simulink model "CNC_pp_obs"  (R2024b)
settings: Solver=VariableStepAuto  StartTime=0.0  StopTime=10.0  RelTol=1e-3
PostLoadFcn:
  | addpath(fileparts(fileparts(get_param(bdroot,'FileName'))));
StartFcn:
  |    addpath(fullfile(fileparts(get_param(bdroot,'FileName')),'..','scripts'));
  |    run_and_save_deferred(bdroot, 'start');
StopFcn:
  |    addpath(fullfile(fileparts(get_param(bdroot,'FileName')),'..','scripts'));
  |    run_and_save_deferred(bdroot, 'stop');
undefined symbols (not defined in the file): A_obs_3165, A_obs_3166, B_obs_3165, B_obs_3166, HIL, k_3165_load, k_3166_load, Kaw_3165, Kaw_3166, kd_3165, kd_3166, ki_3165, Ki_3165, ki_3166, Ki_3166, kp_3165, kp_3166, Kx_3165, Kx_3166, qc_get_step_size, tau_3165_load, tau_3166_load
libraries: quarc_library x4, slpidlib x2
settings Model: Creator=ricca  LastModifiedBy=ricca

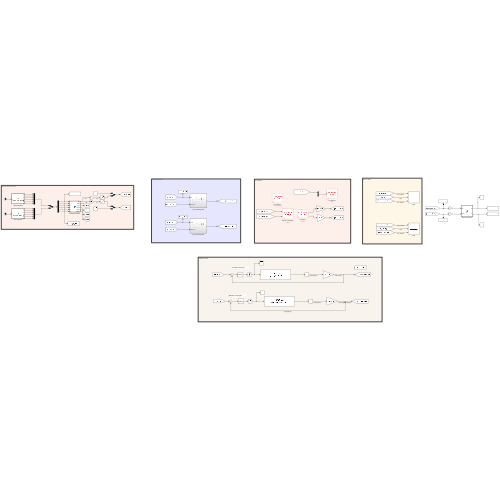
[thumbnail: Simulink's stored preview of the top-level diagram]
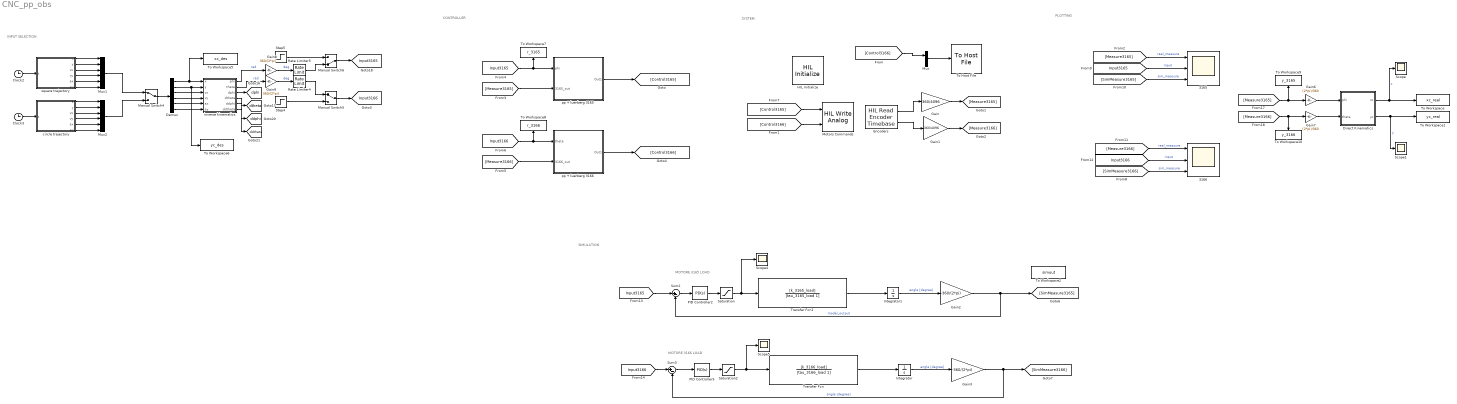
== system CNC_pp_obs ==
  note: MOTORE 3165 LOAD
  note: PLOTTING
  note: CONTROLLER
  note: MOTORE 3166 LOAD
  note: SIMULATION
  note: SYSTEM
  note: INPUT SELECTION
  3165 : Scope  NumInputPorts=3
  3166 : Scope  NumInputPorts=3
  Clock2 : Clock
  Clock3 : Clock
  Demux : Demux  Outputs=6
  Direct Kinematics : MATLAB Function  TreatAsAtomicUnit=on  SystemSampleTime=0.002
  Encoders : quarc_library/Data Acquisition/Generic/Timebases/HIL Read Encoder Timebase  object_name=HIL-1  clock=0  channels=0:1  active=on  vector_output=off  data_type_mode=Inherit via back propagation  data_type=double  overflow_mode=Error on overflow  samples_in_buffer=max(ceil(1/qc_get_step_size), 1)
  Gain : Gain  Gain=360/4096
  Gain1 : Gain  Gain=360/4096
  Gain2 : Gain  Gain=-360/(2*pi)
  Gain3 : Gain  Gain=-360/(2*pi)
  Gain6 : Gain  Gain=(2*pi)/360
  Gain7 : Gain  Gain=(2*pi)/360
  Gain8 : Gain  Gain=360/(2*pi)
  Gain9 : Gain  Gain=360/(2*pi)
  HIL Initialize : quarc_library/Data Acquisition/Generic/Configuration/HIL Initialize  object_name=HIL-1  board_type=q2_usb  board_number=0  board_options=d0=digital;d1=digital;led=auto;update_rate=normal;decimation=1  exclusive=off  active=off  hardware_clocks=[0]  clock_modes=[]  initial_clock_frequencies=[]  set_clock_params_at_start=off  set_clock_params_at_switch_in=off  set_clock_frequencies_at_start=off  set_clock_frequencies_at_switch_in=off  analog_input_channels=[0:1]  analog_input_configurations=[]  analog_input_maximums=10  analog_input_minimums=-10  set_analog_input_params_at_start=on  set_analog_input_params_at_switch_in=off  analog_output_channels=[0:1]  analog_output_maximums=10  analog_output_minimums=-10  initial_analog_outputs=[0]  final_analog_outputs=[0]  watchdog_analog_outputs=0  set_analog_output_params_at_start=on  set_analog_output_params_at_switch_in=off  set_analog_outputs_at_start=on  set_analog_outputs_at_switch_in=off  set_analog_outputs_at_terminate=on  set_analog_outputs_at_switch_out=off  set_analog_outputs_on_watchdog=off  digital_input_channels=[]  digital_output_channels=[]  digital_output_configuration=[]  initial_digital_outputs=[1]  final_digital_outputs=[1]  watchdog_digital_outputs=[1]  set_digital_output_params_at_start=off  set_digital_output_params_at_switch_in=off  set_digital_outputs_at_start=on  set_digital_outputs_at_switch_in=off  set_digital_outputs_at_terminate=on  set_digital_outputs_at_switch_out=off  set_digital_outputs_on_watchdog=off  encoder_channels=[0:1]  quadrature=[4]  encoder_filter_frequency=[]  initial_encoder_counts=[0]  set_encoder_params_at_start=on  set_encoder_params_at_switch_in=off  set_encoder_counts_at_start=on  set_encoder_counts_at_switch_in=off  pwm_channels=[]  pwm_modes=[0]  pwm_frequency=1/0.020  pwm_configuration=[]  pwm_alignment=[]  pwm_polarity=[]  pwm_leading_deadband=[]  pwm_trailing_deadband=[]  initial_pwm_outputs=[0]  final_pwm_outputs=[0]  watchdog_pwm_outputs=[0]  set_pwm_params_at_start=on  set_pwm_params_at_switch_in=off  set_pwm_outputs_at_start=on  set_pwm_outputs_at_switch_in=off  set_pwm_outputs_at_terminate=on  set_pwm_outputs_at_switch_out=off  set_pwm_outputs_on_watchdog=off  other_output_channels=[]  initial_other_outputs=[]  final_other_outputs=[]  watchdog_other_outputs=[]  set_other_outputs_at_start=off  set_other_outputs_at_switch_in=off  set_other_outputs_at_terminate=off  set_other_outputs_at_switch_out=off  set_other_outputs_on_watchdog=off
  Integrator : Integrator
  Integrator1 : Integrator
  Manual Switch4 : ManualSwitch
  Manual Switch5 : ManualSwitch
  Manual Switch6 : ManualSwitch  CurrentSetting=0
  Motors Commands : quarc_library/Data Acquisition/Generic/Immediate I//O/HIL Write Analog  object_name=HIL-1  channels=0:1  sample_time=-1  active=off  vector_input=off
  Mux : Mux  Inputs=2
  Mux1 : Mux  Inputs=6
  Mux2 : Mux  Inputs=6
  PID Controller2 : slpidlib/PID Controller  Controller=PD  Form=Parallel  TimeDomain=Continuous-time  UseExternalTs=off  SampleTime=-1  IntegratorMethod=Forward Euler  FilterMethod=Forward Euler  ControllerParametersSource=internal  P=kp_3165  I=ki_3165  UseKiTs=off  D=kd_3165  UseExternalDerivativeSource=off  N=100  UseFilter=on  TunerSelectOption=Transfer Function Based (PID Tuner App)  InitialConditionSource=internal  InitialConditionForIntegrator=0  InitialConditionForFilter=0  DifferentiatorICPrevScaledInput=0  ExternalReset=none  TrackingMode=off  Kt=1  LimitOutput=off  SatLimitsSource=internal  UpperSaturationLimit=inf  LowerSaturationLimit=-inf  LinearizeAsGain=on  AntiWindupMode=none  Kb=1  LimitIntegrator=off  UpperIntegratorSaturationLimit=inf  LowerIntegratorSaturationLimit=-inf  POutMin=[]  POutMax=[]  IOutMin=[]  IOutMax=[]  DOutMin=[]  DOutMax=[]  NOutMin=[]  NOutMax=[]  SumOutMin=[]  SumOutMax=[]  SaturationOutMin=[]  SaturationOutMax=[]  PParamMin=[]  PParamMax=[]  IParamMin=[]  IParamMax=[]  DParamMin=[]  DParamMax=[]  NParamMin=[]  NParamMax=[]  KbParamMin=[]  KbParamMax=[]  KtParamMin=[]  KtParamMax=[]  KbOutMin=[]  KbOutMax=[]  KtOutMin=[]  KtOutMax=[]  IntegratorOutMin=[]  IntegratorOutMax=[]  FilterOutMin=[]  FilterOutMax=[]  SumI1OutMin=[]  SumI1OutMax=[]  SumI2OutMin=[]  SumI2OutMax=[]  SumI3OutMin=[]  SumI3OutMax=[]  SumI4OutMin=[]  SumI4OutMax=[]  SumDOutMin=[]  SumDOutMax=[]  DifferentiatorOutMin=[]  DifferentiatorOutMax=[]  FilterDiffOutCoefMin=[]  FilterDiffOutCoefMax=[]  ReciprocalOutMin=[]  ReciprocalOutMax=[]  SumDenOutMin=[]  SumDenOutMax=[]  SumNumOutMin=[]  SumNumOutMax=[]  DivideOutMin=[]  DivideOutMax=[]  UdiffTsProdOutMin=[]  UdiffTsProdOutMax=[]  NTsProdOutMin=[]  NTsProdOutMax=[]  UintegralTsProdOutMin=[]  UintegralTsProdOutMax=[]  UngainTsProdOutMin=[]  UngainTsProdOutMax=[]  ClampingZeroOutDataTypeStr=Inherit: Inherit via back propagation  ClampingZeroOutMin=[]  ClampingZeroOutMax=[]  FilterDenConstantOutDataTypeStr=Inherit: Inherit via back propagation  FilterDenConstantOutMin=[]  FilterDenConstantOutMax=[]  PCopyOutDataTypeStr=Inherit: Inherit via back propagation  PCopyOutMin=[]  PCopyOutMax=[]  NCopyOutDataTypeStr=Inherit: Inherit via back propagation  NCopyOutMin=[]  NCopyOutMax=[]  IntegratorContinuousStateAttributes=''  IntegratorStateMustResolveToSignalObject=off  IntegratorRTWStateStorageClass=Auto  FilterContinuousStateAttributes=''  FilterStateMustResolveToSignalObject=off  FilterRTWStateStorageClass=Auto  ParallelPVariant=InternalParameters  IdealPVariant=Disabled  IVariant=Disabled  DVariant=InternalParameters  IntegratorVariant=Disabled  SatVariant=Disabled  AWVariant=Disabled  PCopyVariant=Disabled  TRVariant=Disabled  FdbkBlocksVariant=Forward  IdealPFdbkVariant=Disabled  SatFdbkVariant=Disabled  DerivativeFilterVariant=ContFilter  NVariant=InternalParameters  NCopyVariant=Disabled  FilterICVariant=InternalICsFilter  IntegratorICVariant=Disabled  ExternalResetVariant=Disabled  TRSumVariant=Passthrough  SumFdbkVariant=Disabled  SumVariant=Sum_PD  TsampFilterVariant=InternalTs  TsampNgainVariant=Passthrough  TsampIntegralVariant=Disabled_SignalSpec  ExternalSaturationOutDataTypeStr=Inherit: Same as second input  DerivativeSourceVariant=ErrorSignal  PreIntVariant=InternalPreInt
  PID Controller3 : slpidlib/PID Controller  Controller=PID  Form=Parallel  TimeDomain=Continuous-time  UseExternalTs=off  SampleTime=-1  IntegratorMethod=Forward Euler  FilterMethod=Forward Euler  ControllerParametersSource=internal  P=kp_3166  I=ki_3166  UseKiTs=off  D=kd_3166  UseExternalDerivativeSource=off  N=100  UseFilter=on  TunerSelectOption=Transfer Function Based (PID Tuner App)  InitialConditionSource=internal  InitialConditionForIntegrator=0  InitialConditionForFilter=0  DifferentiatorICPrevScaledInput=0  ExternalReset=none  TrackingMode=off  Kt=1  LimitOutput=off  SatLimitsSource=internal  UpperSaturationLimit=inf  LowerSaturationLimit=-inf  LinearizeAsGain=on  AntiWindupMode=none  Kb=1  LimitIntegrator=off  UpperIntegratorSaturationLimit=inf  LowerIntegratorSaturationLimit=-inf  POutMin=[]  POutMax=[]  IOutMin=[]  IOutMax=[]  DOutMin=[]  DOutMax=[]  NOutMin=[]  NOutMax=[]  SumOutMin=[]  SumOutMax=[]  SaturationOutMin=[]  SaturationOutMax=[]  PParamMin=[]  PParamMax=[]  IParamMin=[]  IParamMax=[]  DParamMin=[]  DParamMax=[]  NParamMin=[]  NParamMax=[]  KbParamMin=[]  KbParamMax=[]  KtParamMin=[]  KtParamMax=[]  KbOutMin=[]  KbOutMax=[]  KtOutMin=[]  KtOutMax=[]  IntegratorOutMin=[]  IntegratorOutMax=[]  FilterOutMin=[]  FilterOutMax=[]  SumI1OutMin=[]  SumI1OutMax=[]  SumI2OutMin=[]  SumI2OutMax=[]  SumI3OutMin=[]  SumI3OutMax=[]  SumI4OutMin=[]  SumI4OutMax=[]  SumDOutMin=[]  SumDOutMax=[]  DifferentiatorOutMin=[]  DifferentiatorOutMax=[]  FilterDiffOutCoefMin=[]  FilterDiffOutCoefMax=[]  ReciprocalOutMin=[]  ReciprocalOutMax=[]  SumDenOutMin=[]  SumDenOutMax=[]  SumNumOutMin=[]  SumNumOutMax=[]  DivideOutMin=[]  DivideOutMax=[]  UdiffTsProdOutMin=[]  UdiffTsProdOutMax=[]  NTsProdOutMin=[]  NTsProdOutMax=[]  UintegralTsProdOutMin=[]  UintegralTsProdOutMax=[]  UngainTsProdOutMin=[]  UngainTsProdOutMax=[]  ClampingZeroOutDataTypeStr=Inherit: Inherit via back propagation  ClampingZeroOutMin=[]  ClampingZeroOutMax=[]  FilterDenConstantOutDataTypeStr=Inherit: Inherit via back propagation  FilterDenConstantOutMin=[]  FilterDenConstantOutMax=[]  PCopyOutDataTypeStr=Inherit: Inherit via back propagation  PCopyOutMin=[]  PCopyOutMax=[]  NCopyOutDataTypeStr=Inherit: Inherit via back propagation  NCopyOutMin=[]  NCopyOutMax=[]  IntegratorContinuousStateAttributes=''  IntegratorStateMustResolveToSignalObject=off  IntegratorRTWStateStorageClass=Auto  FilterContinuousStateAttributes=''  FilterStateMustResolveToSignalObject=off  FilterRTWStateStorageClass=Auto  ParallelPVariant=InternalParameters  IdealPVariant=Disabled  IVariant=InternalParameters  DVariant=InternalParameters  IntegratorVariant=Continuous  SatVariant=Disabled  AWVariant=Passthrough  PCopyVariant=Disabled  TRVariant=Disabled  FdbkBlocksVariant=Forward  IdealPFdbkVariant=Disabled  SatFdbkVariant=Disabled  DerivativeFilterVariant=ContFilter  NVariant=InternalParameters  NCopyVariant=Disabled  FilterICVariant=InternalICsFilter  IntegratorICVariant=InternalICs  ExternalResetVariant=Disabled  TRSumVariant=Passthrough  SumFdbkVariant=Disabled  SumVariant=Sum_PID  TsampFilterVariant=InternalTs  TsampNgainVariant=Passthrough  TsampIntegralVariant=Disabled_SignalSpec  ExternalSaturationOutDataTypeStr=Inherit: Same as second input  DerivativeSourceVariant=ErrorSignal  PreIntVariant=InternalPreInt
  Rate Limiter4 : RateLimiter  RisingSlewLimit=100  FallingSlewLimit=-100  SampleTimeMode=inherited
  Rate Limiter5 : RateLimiter  RisingSlewLimit=100  FallingSlewLimit=-100  SampleTimeMode=inherited
  Saturation : Saturate  UpperLimit=6  LowerLimit=-6
  Saturation2 : Saturate  UpperLimit=6  LowerLimit=-6
  Scope{,1,4..5} (4 alike) : Scope
  Step4 : Step  After=10  SampleTime=0
  Step5 : Step  After=10  SampleTime=0
  Sum2 : Sum  Inputs=|+-
  Sum3 : Sum  Inputs=|+-
  To Host File : quarc_library/Sinks/To Host/To Host File  source=Specify via dialog (do not evaluate)  file_name=data_%{date}_%{time}.mat  variable_name=data  decimation=1  sample_time=-1  file_format=MAT-file v.4  options=No header or footer  append=off  final_file_name=data_19-Oct-2026_18-54-36.mat  encoding=Default  bitrate=2000000
  To Workspace : ToWorkspace  VariableName=xc_real  SampleTime=-1
  To Workspace1 : ToWorkspace  VariableName=yc_real  SampleTime=-1
  To Workspace10 : ToWorkspace  VariableName=y_3166  SaveFormat=Timeseries  SampleTime=0.002
  To Workspace2 : ToWorkspace  VariableName=simout  SaveFormat=Timeseries  SampleTime=-1
  To Workspace5 : ToWorkspace  VariableName=xc_des  SaveFormat=Timeseries  SampleTime=0.002
  To Workspace6 : ToWorkspace  VariableName=yc_des  SaveFormat=Timeseries  SampleTime=0.002
  To Workspace7 : ToWorkspace  VariableName=r_3165  SaveFormat=Timeseries  SampleTime=0.002
  To Workspace8 : ToWorkspace  VariableName=r_3166  SaveFormat=Timeseries  SampleTime=0.002
  To Workspace9 : ToWorkspace  VariableName=y_3165  SaveFormat=Timeseries  SampleTime=0.002
  Transfer Fcn : TransferFcn  Numerator=[k_3166_load]  Denominator=[tau_3166_load 1]
  Transfer Fcn1 : TransferFcn  Numerator=[k_3165_load]  Denominator=[tau_3165_load 1]
  circle trajectory : MATLAB Function  TreatAsAtomicUnit=on
  inverse kinematics : MATLAB Function  TreatAsAtomicUnit=on  SystemSampleTime=0.002
  pp + luenberg 3165 : Subsystem
  pp + luenberg 3166 : Subsystem
  square trajectory : MATLAB Function  TreatAsAtomicUnit=on
  tag scope: Input3165=global, Input3166=global, ddphi=global, ddtheta=global, dphi=global, dtheta=global
  wires:
  Encoders/1 -> Gain/1
  [Control3166] -> Motors Commands/2
  Direct Kinematics/2(yc) -> Scope1/1, To Workspace1/1  "y"
  Gain6/1 -> Direct Kinematics/1(phi)
  [Measure3166] -> 3166/1  "real_measure"
  [SimMeasure3165] -> 3165/3  "sim_measure"
  PID Controller3/1 -> Saturation2/1
  Gain7/1 -> Direct Kinematics/2(theta)
  [Input3165] -> pp + luenberg 3165/1(phi), To Workspace7/1
  [Input3165] -> Sum2/1
  Sum3/1 -> PID Controller3/1
  Integrator1/1 -> Gain2/1  "angle [degree]"
  [SimMeasure3166] -> 3166/3  "sim_measure"
  Transfer Fcn/1 -> Integrator/1
  Gain3/1 -> [SimMeasure3166], Sum3/2  "angle [degree]"
  Sum2/1 -> PID Controller2/1
  [Control3165] -> Motors Commands/1
  [Measure3165] -> Gain6/1, To Workspace9/1
  Integrator/1 -> Gain3/1  "angle [degree]"
  [Measure3166] -> To Workspace10/1, Gain7/1
  Gain1/1 -> [Measure3166]
  [Input3166] -> 3166/2  "input"
  [Control3166] -> Mux/1
  [Input3165] -> 3165/2  "input"
  Gain/1 -> [Measure3165]
  [Measure3165] -> pp + luenberg 3165/2(3165_out)
  Saturation2/1 -> Scope5/1, Transfer Fcn/1
  Encoders/2 -> Gain1/1
  Gain2/1 -> [SimMeasure3165], Sum2/2  "model_output"
  [Input3166] -> Sum3/1
  Direct Kinematics/1(xc) -> To Workspace/1, Scope/1  "x"
  [Measure3166] -> pp + luenberg 3166/2(3166_out)
  [Measure3165] -> 3165/1  "real_measure"
  PID Controller2/1 -> Saturation/1
  pp + luenberg 3165/1(Out1) -> [Control3165]
  Saturation/1 -> Scope4/1, Transfer Fcn1/1
  [Input3166] -> pp + luenberg 3166/1(theta), To Workspace8/1
  Transfer Fcn1/1 -> Integrator1/1
  Mux/1 -> To Host File/1
  pp + luenberg 3166/1(Out1) -> [Control3166]
  Manual Switch5/1 -> [Input3166]
  circle trajectory/6(ay) -> Mux2/6
  Clock3/1 -> circle trajectory/1(t)
  Manual Switch6/1 -> [Input3165]
  Demux/1 -> inverse kinematics/1(x), To Workspace5/1
  Mux2/1 -> Manual Switch4/2
  square trajectory/2(y) -> Mux1/2
  Rate Limiter5/1 -> Manual Switch6/2
  inverse kinematics/3(dphi) -> [dphi]
  square trajectory/1(x) -> Mux1/1
  Clock2/1 -> square trajectory/1(t)
  inverse kinematics/2(theta) -> Gain9/1  "rad"
  Rate Limiter4/1 -> Manual Switch5/1
  square trajectory/6(ay) -> Mux1/6
  circle trajectory/2(y) -> Mux2/2
  inverse kinematics/4(dtheta) -> [dtheta]
  Demux/5 -> inverse kinematics/5(ax)
  Step4/1 -> Manual Switch5/2
  circle trajectory/3(vx) -> Mux2/3
  Mux1/1 -> Manual Switch4/1
  inverse kinematics/1(phi) -> Gain8/1  "rad"
  circle trajectory/4(vy) -> Mux2/4
  Demux/2 -> To Workspace6/1, inverse kinematics/2(y)
  inverse kinematics/5(ddphi) -> [ddphi]
  circle trajectory/5(ax) -> Mux2/5
  inverse kinematics/6(ddtheta) -> [ddtheta]
  Gain9/1 -> Rate Limiter4/1  "deg"
  Manual Switch4/1 -> Demux/1
  square trajectory/4(vy) -> Mux1/4
  Demux/4 -> inverse kinematics/4(vy)
  Step5/1 -> Manual Switch6/1
  Demux/6 -> inverse kinematics/6(ay)
  Gain8/1 -> Rate Limiter5/1  "deg"
  Demux/3 -> inverse kinematics/3(vx)
  square trajectory/5(ax) -> Mux1/5
  square trajectory/3(vx) -> Mux1/3
  circle trajectory/1(x) -> Mux2/1

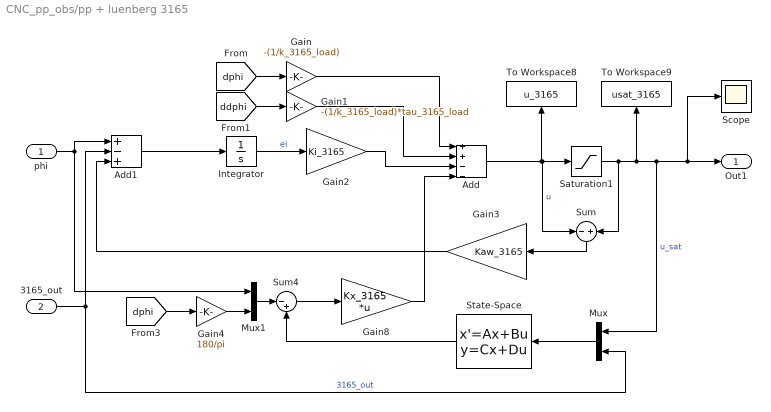
== system CNC_pp_obs/pp + luenberg 3165 ==
  phi : Inport
  3165_out : Inport  Port=2
  Add : Sum  Inputs=++--
  Add1 : Sum  Inputs=+-+
  Gain : Gain  Gain=-(1/k_3165_load)
  Gain1 : Gain  Gain=-(1/k_3165_load)*tau_3165_load
  Gain2 : Gain  Gain=Ki_3165
  Gain3 : Gain  Gain=Kaw_3165
  Gain4 : Gain  Gain=180/pi
  Gain8 : Gain  Gain=Kx_3165  Multiplication=Matrix(K*u)
  Integrator : Integrator
  Mux : Mux  Inputs=2
  Mux1 : Mux  Inputs=2
  Saturation1 : Saturate  UpperLimit=6  LowerLimit=-6
  Scope : Scope
  State-Space : StateSpace  A=A_obs_3165  B=B_obs_3165  C=eye(2)  D=zeros(2,2)  InitialCondition=0
  Sum : Sum  Inputs=-|+
  Sum4 : Sum  Inputs=|-+
  To Workspace8 : ToWorkspace  VariableName=u_3165  SaveFormat=Timeseries  SampleTime=0.002
  To Workspace9 : ToWorkspace  VariableName=usat_3165  SaveFormat=Timeseries  SampleTime=0.002
  Out1 : Outport
  wires:
  3165_out/1 -> Mux/2, Add1/2  "3165_out"
  [dphi] -> Gain/1
  Gain/1 -> Add/1
  [ddphi] -> Gain1/1
  Add/1 -> Sum/1, Saturation1/1, To Workspace8/1  "u"
  Saturation1/1 -> Sum/2, To Workspace9/1, Scope/1, Out1/1, Mux/1  "u_sat"
  Sum4/1 -> Gain8/1
  State-Space/1 -> Sum4/2
  Mux/1 -> State-Space/1
  phi/1 -> Add1/1, Mux1/1
  Integrator/1 -> Gain2/1  "ei"
  Mux1/1 -> Sum4/1
  Gain1/1 -> Add/2
  Gain8/1 -> Add/4
  Gain2/1 -> Add/3
  Sum/1 -> Gain3/1
  Add1/1 -> Integrator/1
  Gain3/1 -> Add1/3
  [dphi] -> Gain4/1
  Gain4/1 -> Mux1/2

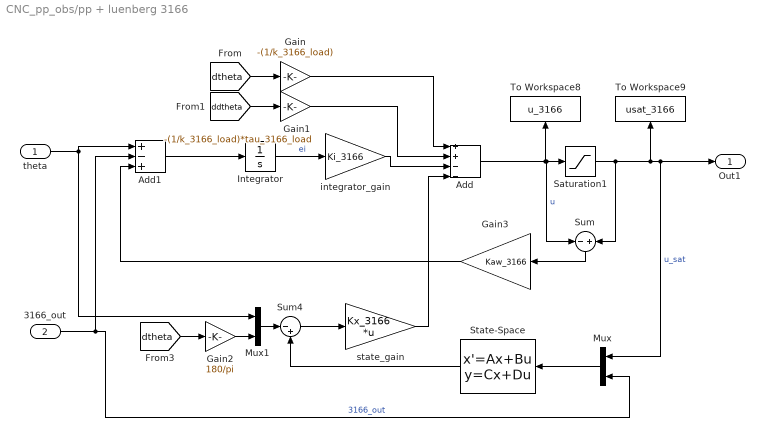
== system CNC_pp_obs/pp + luenberg 3166 ==
  theta : Inport
  3166_out : Inport  Port=2
  Add : Sum  Inputs=++--
  Add1 : Sum  Inputs=+-+
  Gain : Gain  Gain=-(1/k_3166_load)
  Gain1 : Gain  Gain=-(1/k_3166_load)*tau_3166_load
  Gain2 : Gain  Gain=180/pi
  Gain3 : Gain  Gain=Kaw_3166
  Integrator : Integrator
  Mux : Mux  Inputs=2
  Mux1 : Mux  Inputs=2
  Saturation1 : Saturate  UpperLimit=6  LowerLimit=-6
  State-Space : StateSpace  A=A_obs_3166  B=B_obs_3166  C=eye(2)  D=zeros(2,2)  InitialCondition=0
  Sum : Sum  Inputs=-|+
  Sum4 : Sum  Inputs=|-+
  To Workspace8 : ToWorkspace  VariableName=u_3166  SaveFormat=Timeseries  SampleTime=0.002
  To Workspace9 : ToWorkspace  VariableName=usat_3166  SaveFormat=Timeseries  SampleTime=0.002
  integrator_gain : Gain  Gain=Ki_3166
  state_gain : Gain  Gain=Kx_3166  Multiplication=Matrix(K*u)
  Out1 : Outport
  wires:
  3166_out/1 -> Add1/2, Mux/2  "3166_out"
  [dtheta] -> Gain/1
  Gain/1 -> Add/1
  [ddtheta] -> Gain1/1
  Sum4/1 -> state_gain/1
  State-Space/1 -> Sum4/2
  Mux/1 -> State-Space/1
  theta/1 -> Mux1/1, Add1/1
  Integrator/1 -> integrator_gain/1  "ei"
  Mux1/1 -> Sum4/1
  Gain1/1 -> Add/2
  state_gain/1 -> Add/4
  integrator_gain/1 -> Add/3
  Sum/1 -> Gain3/1
  Add/1 -> Saturation1/1, Sum/1, To Workspace8/1  "u"
  Saturation1/1 -> Sum/2, To Workspace9/1, Mux/1, Out1/1  "u_sat"
  Add1/1 -> Integrator/1
  Gain3/1 -> Add1/3
  [dtheta] -> Gain2/1
  Gain2/1 -> Mux1/2

== matlab function CNC_pp_obs/Direct Kinematics ==
  data: phi input; xc output; theta input; yc output
function [xc, yc] = fcn(phi, theta)
l = 0.127;
a = 2 - sin(theta) - cos(phi);
b = cos(theta) - sin(phi);
s = sqrt(a^2 + b^2);
h = l*sqrt(1 - s^2/4);

% Nonlinear forward kinematics of point C
xc = l/2*(2 - sin(theta) + cos(phi)) - h*b/s;
yc = l/2*(cos(theta) + sin(phi))     + h*a/s;

== matlab function CNC_pp_obs/square trajectory ==
  data: x output; t input; y output; vx output; vy output; ax output; ay output
function [x, y, vx, vy, ax, ay] = square_gen_smooth(t)
c  = [0.127; 0.127];
s  = 0.09;
T  = 4;
Ts = T/4;
P = [c(1)-s/2, c(1)+s/2, c(1)+s/2, c(1)-s/2, c(1)-s/2;
     c(2)-s/2, c(2)-s/2, c(2)+s/2, c(2)+s/2, c(2)-s/2];

tau = mod(t, T) / Ts;
k   = min(floor(tau), 3);
f   = tau - k;

% quintic time scaling and its derivatives w.r.t. real time
sig   = 10*f^3 - 15*f^4 + 6*f^5;
dsig  = (30*f^2 - 60*f^3 + 30*f^4) / Ts;
ddsig = (60*f - 180*f^2 + 120*f^3) / Ts^2;

dx = P(1,k+2) - P(1,k+1);
dy = P(2,k+2) - P(2,k+1);

x  = P(1,k+1) + sig*dx;     y  = P(2,k+1) + sig*dy;
vx = dsig*dx;               vy = dsig*dy;
ax = ddsig*dx;              ay = ddsig*dy;
end

== matlab function CNC_pp_obs/circle trajectory ==
  data: x output; t input; y output; vx output; vy output; ax output; ay output
function [x, y, vx, vy, ax, ay] = circle_gen_smooth(t)
% The circle is inscribed in the square (same center, diameter = side).
c   = [0.127; 0.127];   % center [m]
s   = 0.09;             % side of the square [m]
r   = s/2;              % radius [m]
T   = 4;                % duration of one lap [s]
th0 = 5*pi/4;           % starting angle: bottom-left, like the square

% quintic time scaling on the angle: one full lap in T seconds,
% with zero velocity and acceleration at the start and end of each lap
f     = mod(t, T) / T;                              % normalized time 0..1
sig   = 10*f^3 - 15*f^4 + 6*f^5;
dsig  = (30*f^2 - 60*f^3 + 30*f^4) / T;
ddsig = (60*f - 180*f^2 + 120*f^3) / T^2;

th   = th0 + 2*pi*sig;      % angle on the circle [rad]
dth  = 2*pi*dsig;           % angular velocity [rad/s]
ddth = 2*pi*ddsig;          % angular acceleration [rad/s^2]

% position, velocity and acceleration (chain rule)
x  = c(1) + r*cos(th);
y  = c(2) + r*sin(th);
vx = -r*sin(th)*dth;
vy =  r*cos(th)*dth;
ax = -r*cos(th)*dth^2 - r*sin(th)*ddth;   % centripetal + tangential
ay = -r*sin(th)*dth^2 + r*cos(th)*ddth;
end

== matlab function CNC_pp_obs/inverse kinematics ==
  data: x input; phi output; y input; theta output; vx input; vy input; ax input; ay input; dphi output; dtheta output; ddphi output; ddtheta output
function [phi, theta, dphi, dtheta, ddphi, ddtheta] = fcn(x, y, vx, vy, ax, ay)
% Inverse kinematics + joint velocity/acceleration, self-contained.
l = 0.127;

persistent q0
if isempty(q0)
    q0 = [0; 0];                 % home configuration
end

% ---- position IK (damped Newton, warm-started from previous step) ----
q = q0;
p_des   = [x; y];
maxIter = 50;
tol     = 1e-9;
lambda  = 1e-10;
for k = 1:maxIter
    p   = FK(q(1), q(2), l);
    err = p - p_des;
    if norm(err) < tol
        break
    end
    J  = jac(q, l);
    dq = -(J.'*J + lambda*eye(2)) \ (J.'*err);
    st = 1;
    for m = 1:10
        qn = q + st*dq;
        if norm(FK(qn(1), qn(2), l) - p_des) < norm(err)
            break
        end
        st = st/2;
    end
    q = q + st*dq;
end
q0 = q;                          % warm start for next call
phi   = q(1);
theta = q(2);

% ---- velocity and acceleration ----
J  = jac(q, l);
qd = J \ [vx; vy];

e    = 1e-4;
Jdot = (jac(q + e*qd, l) - jac(q - e*qd, l)) / (2*e);
qdd  = J \ ([ax; ay] - Jdot*qd);

dphi   = qd(1);   dtheta  = qd(2);
ddphi  = qdd(1);  ddtheta = qdd(2);
end

function J = jac(q, l)
h = 1e-6;
J = zeros(2,2);
for j = 1:2
    d = zeros(2,1);
    d(j) = h;
    J(:,j) = (FK(q(1)+d(1), q(2)+d(2), l) - FK(q(1)-d(1), q(2)-d(2), l)) / (2*h);
end
end

function p = FK(phi, theta, l)
a = 2 - sin(theta) - cos(phi);
b = cos(theta) - sin(phi);
s = sqrt(a^2 + b^2);
s = max(s, 1e-9);
h = l * sqrt(max(1 - s^2/4, 0));
xc = l/2*(2 - sin(theta) + cos(phi)) - h*b/s;
yc = l/2*(cos(theta) + sin(phi))     + h*a/s;
p  = [xc; yc];
end
